simulink subsystem "Yaw_Scopes"  (R2025a)
settings: Solver=VariableStepAuto  StartTime=0.0  StopTime=10.0  RelTol=1e-3
Description:
  | Copyright 2025 The MathWorks, Inc.
settings Model: Creator=smiller  LastModifiedBy=smiller

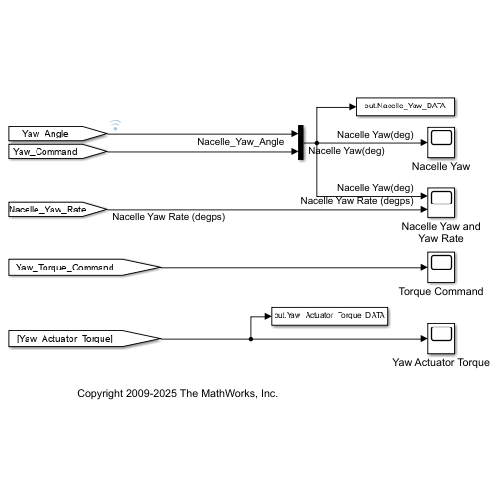
[thumbnail: Simulink's stored preview of the top-level diagram]
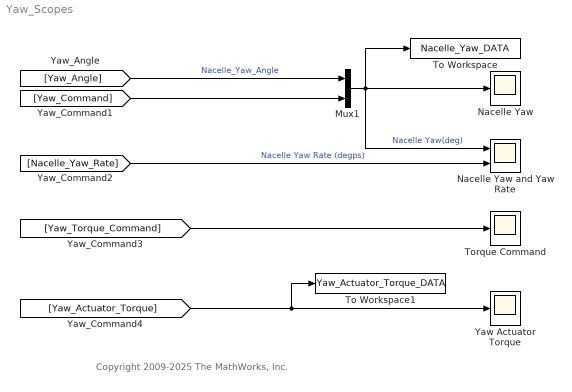
== system Yaw_Scopes ==
  note: Copyright 2009-2025 The MathWorks, Inc.
  Mux1 : Mux  Inputs=2
  Nacelle Yaw : Scope
      settings: TimeSpan=80  ActiveDisplayYMinimum=-4.9099  ActiveDisplayYMaximum=3.7678  DataLoggingVariableName=Nacelle_Yaw_DATA
  Nacelle Yaw and Yaw Rate : Scope  NumInputPorts=2
      settings: TimeSpan=80  ActiveDisplayYMinimum=-5  ActiveDisplayYMaximum=5  DataLoggingVariableName=ScopeData2
  To Workspace : ToWorkspace  VariableName=Nacelle_Yaw_DATA  SaveFormat=Structure With Time  SampleTime=-1
  To Workspace1 : ToWorkspace  VariableName=Yaw_Actuator_Torque_DATA  SaveFormat=Structure With Time  SampleTime=-1
  Torque Command : Scope
      settings: TimeSpan=3.951473136915078  DataLoggingVariableName=ScopeData3
  Yaw Actuator Torque : Scope
      settings: ActiveDisplayYMinimum=-287.2251  ActiveDisplayYMaximum=274.1131  DataLoggingVariableName=Yaw_Actuator_Torque_DATA
  wires:
  Mux1/1 -> Nacelle Yaw/1, To Workspace/1, Nacelle Yaw and Yaw Rate/1  "Nacelle Yaw(deg)"
  [Yaw_Actuator_Torque] -> To Workspace1/1, Yaw Actuator Torque/1
  [Yaw_Command] -> Mux1/2
  [Yaw_Torque_Command] -> Torque Command/1
  [Yaw_Angle] -> Mux1/1  "Nacelle_Yaw_Angle"
  [Nacelle_Yaw_Rate] -> Nacelle Yaw and Yaw Rate/2  "Nacelle Yaw Rate (degps)"
